simulink model "EMT_ML.before_diagnostic_fixes"  (R2024b)
settings: Solver=ode5  StartTime=0.0  StopTime=200  FixedStep=0.002  RelTol=1e-3
model workspace (MAT data in the model file):
  A = 7.3
  B = 2.71
  C0_shift = 200
  C1_shift = 200
  C2_shift = 200
  Cb = 70
  Cd = 0.6
  EMSInputBus : Simulink.Bus (value not decoded)
  Fb_max = 247500
  JA = 0.4
  JB = 0.4
  JZ = 0.4
  Jc1r2 = 0.01
  Jc3r4 = 0.01
  Jc4 = 0.01
  Je = 2.5
  Jh = 0.01
  Jq1 = 0.01
  Jq2 = 0.01
  Jr1 = 0.01
  Jr3s4 = 0.01
  Js123 = 0.01
  L = 4.472
  NE = [1600 1600 1600 1600 1600 1600 1600 1600 1600 1600 1600 1600 ... (840 elements, 30x28)]
  N_Te = 30
  N_ne = 28
  PE = [0 100.366530527 133.710336161 167.221698607 195.706356687 221.845219395 250.497434286 278.144308305 305.288511886 330.086920096 352.87464656 374.489475338 ... (840 elements, 30x28)]
  PN0 = 0
  Pb_epr = [-45 -45 -40 -30 0 30 40 45 45]
  Pb_max = [0 40 45 45 45]
  Pb_min = [-45 -45 -45 -40 0]
  Pe_ass = 230
  Pe_max = 1103
  Peg = [0 100 120 140 160 180 200 220 240 260 280 300 ... (53 elements, 1x53)]
  R_map = [0.09 0.089 0.09 0.091 0.092 0.093 0.094 0.095 0.096 0.097 0.098]
  SF_C0 = 1.5
  SF_C1 = 1.5
  SF_C2 = 1.5
  SF_Z1 = 1.5
  SF_Z2 = 1.5
  SF_ZD = 1.5
  SOC0 = 60
  SOC_epr = [30 31 50 59 60 61 70 79 80]
  SOC_map = [0 10 20 30 40 50 60 70 80 90 100]
  TA_max_map = [588.855 593.803361345 598.83559322 603.953846154 609.160344828 614.457391304 619.847368421 625.332743363 630.916071429 636.6 642.387272727 648.280733945 ... (115 elements, 1x115)]
  TA_min_map = [-588.855 -593.803361345 -598.83559322 -603.953846154 -609.160344828 -614.457391304 -619.847368421 -625.332743363 -630.916071429 -636.6 -642.387272727 -648.280733945 ... (115 elements, 1x115)]
  TAf = 0
  TB_max_map = [588.855 593.803361345 598.83559322 603.953846154 609.160344828 614.457391304 619.847368421 625.332743363 630.916071429 636.6 642.387272727 648.280733945 ... (115 elements, 1x115)]
  TB_min_map = [-588.855 -593.803361345 -598.83559322 -603.953846154 -609.160344828 -614.457391304 -619.847368421 -625.332743363 -630.916071429 -636.6 -642.387272727 -648.280733945 ... (115 elements, 1x115)]
  TBf = 0
  TE = [0 599 798 998 1168 1324 1495 1660 1822 1970 2106 2235 ... (840 elements, 30x28)]
  TS_A = 0.2
  TS_B = 0.2
  TS_C0 = 0.2
  TS_C1 = 0.2
  TS_C2 = 0.2
  TS_Z = 0.2
  TS_Z1 = 0.2
  TS_Z2 = 0.2
  TS_ZD = 0.2
  TZ_max_map = [537.13125 540.509433962 543.930379747 547.394904459 550.903846154 554.458064516 558.058441558 561.705882353 565.401315789 569.145695364 572.94 576.785234899 ... (131 elements, 1x131)]
  TZ_min_map = [-537.13125 -540.509433962 -543.930379747 -547.394904459 -550.903846154 -554.458064516 -558.058441558 -561.705882353 -565.401315789 -569.145695364 -572.94 -576.785234899 ... (131 elements, 1x131)]
  TZf = 0
  T_generator = [0 185 493.333333333 801.666666667 1110 1418.33333333 1726.66666667]
  T_motor = [0 185 493.333333333 801.666666667 1110 1418.33333333 1726.66666667]
  Te_map = [0 599 798 998 1168 1324 1495 1660 1822 1970 2106 2235 ... (30 elements, 1x30)]
  Te_max = 2754
  Te_max_map = [1168 1324 1495 1660 1822 1970 2106 2235 2355 2458 2543 2606 ... (28 elements, 1x28)]
  Te_start = 1600
  Tef = 100
  Teg = [0 596.8125 636.6 718.741935484 799.916230366 859.41 954.422788606 954.9 996.417391304 1078.98305085 1114.05 1169.26530612 ... (53 elements, 1x53)]
  Temax = 998
  Time = [0 0.1 0.2 0.3 0.4 0.5 0.6 0.7 0.8 0.9 1 1.1 ... (2001 elements, 1x2001)]
  Time_ele = [0 4 8 12 16 20 24 28 32 36 40 44 ... (401 elements, 1x401)]
  Time_fg = [0 2 4 6 8 10 12 14 16 18 20 22 ... (801 elements, 1x801)]
  Tmax_C0 = 2754
  Tmax_C1 = 3505.25455609
  Tmax_C2 = 3505.25455609
  Tmax_Z1 = 5584.80955498
  Tmax_Z2 = 16307.6439005
  Tmax_ZD = 3855.6
  Ts_e = 0.1
  Uoc_map = [814.5 917 933.25 945.75 958.25 969.25 978 985.25 993.25 1003.25 1050]
  V_Shift12 = 32
  V_Shift21 = 25
  V_Start = 10
  Voltage0 = 900
  Voltage_epr = [750 760 900 1000 1050]
  Y_engine = 0.955
  Yc = 0.98
  Yh = 0.96
  Yo = 0.92
  Yq = 0.94
  Z1_shift = 200
  Z2_shift = 200
  a11 = 1.54241568346
  a11_L = 1.54241568346
  a12 = -3.86074191629
  a12_L = 2.43173643789
  a21 = -1.04963112005
  a22 = 2.46948356808
  b11 = 0
  b11_L = 0
  b12 = 3.33
  b12_L = 7.8036
  b21 = 2.23571428571
  b22 = -2.13
  c11 = -0.648333656565
  c12 = 0
  c21 = -0.648333656565
  c22 = 0.680511182109
  controller_id = 1
  controller_name = 'Existing heuristic-grid EMS'
  cycle_grade = [0 0 0 0 0 0 0 0 0 0 0 0 ... (2001 elements, 1x2001)]
  cycle_road = [0.045 0.045 0.045 0.045 0.045 0.045 0.045 0.045 0.045 0.045 0.045 0.045 ... (2001 elements, 1x2001)]
  cycle_steering = [0 0 0 0 0 0 0 0 0 0 0 0 ... (2001 elements, 1x2001)]
  cycle_time = [0 0.1 0.2 0.3 0.4 0.5 0.6 0.7 0.8 0.9 1 1.1 ... (2001 elements, 1x2001)]
  d11 = -0.751666343435
  d12 = 0.3003003003
  d21 = -0.751666343435
  d22 = 0.319488817891
  e11 = -1.54241568346
  e12 = 0
  e21 = 1.04963112005
  e22 = -2.23571428571
  eff_generator = [0.8 0.8 0.79 0.79 0.76 0.74 0.72 0.8 0.85 0.88 0.85 0.8 ... (84 elements, 7x12)]
  eff_motor = [0.8 0.8 0.79 0.79 0.76 0.74 0.72 0.8 0.85 0.88 0.85 0.8 ... (84 elements, 7x12)]
  ele_map = [10 11.46 14.13 19.24 20.94 23.21 20.29 20.23 22.28 17.66 16.24 18.95 ... (401 elements, 1x401)]
  ems_runtime_config : object (value not decoded)
  f11 = -3.86074191629
  f12 = 3.33
  f21 = 2.46948356808
  f22 = -2.13
  fg = 0.045
  fg_map = [0.0125 0.0215 0.0332 0.0452 0.0525 0.0589 0.0584 0.0592 0.0621 0.0576 0.055 0.0572 ... (801 elements, 1x801)]
  fuel_gpkwh = [269.874826377 269.874826377 260.084605263 254.895150301 249.802821062 244.062054381 234.972466555 226.630558735 223.93243551 227.612775381 231.379615385 228.983738255 ... (840 elements, 30x28)]
  fuel_map = [269.874826377 269.874826377 260.084605263 254.895150301 249.802821062 244.062054381 234.972466555 226.630558735 223.93243551 227.612775381 231.379615385 228.983738255 ... (840 elements, 30x28)]
  fuel_map_N = [269.874826377 269.874826377 260.084605263 254.895150301 249.802821062 nan nan nan nan nan nan nan ... (840 elements, 30x28)]
  i = 28
  ic = 4.42
  iq = 1.4
  it = 4
  j = 30
  k1 = 2.13
  k2 = 2.13
  k3 = 2.33
  k4 = 1.92
  kh = 2.88
  kq = 2.17
  kt = 1.83
  mass = 45000
  miu_max = 0.8
  nA_map = [-6000 -5950 -5900 -5850 -5800 -5750 -5700 -5650 -5600 -5550 -5500 -5450 ... (115 elements, 1x115)]
  nA_max = 6000
  nA_min = -6000
  nB_map = [-6000 -5950 -5900 -5850 -5800 -5750 -5700 -5650 -5600 -5550 -5500 -5450 ... (115 elements, 1x115)]
  nB_max = 6000
  nB_min = -6000
  nB_start = 0
  nZ_map = [-8000 -7950 -7900 -7850 -7800 -7750 -7700 -7650 -7600 -7550 -7500 -7450 ... (131 elements, 1x131)]
  nZ_max = 8000
  nZ_min = -8000
  n_generator = [0 318.5 796.25 1274 1751.75 2229.5 2707.25 3185 3662.75 4140.5 4618.25 7007]
  n_motor = [0 318.5 796.25 1274 1751.75 2229.5 2707.25 3185 3662.75 4140.5 4618.25 7007]
  ne_idl = 3000
  ne_map = [1600 1700 1800 1900 2000 2100 2200 2300 2400 2500 2600 2700 ... (28 elements, 1x28)]
  ne_max = 4200
  ne_min = 1600
  ne_start = 200
  neg = [1600 1600 1800 1860 1910 2000 2001 2200 2300 2301 2400 2450 ... (53 elements, 1x53)]
  no_Shift12 = 1589.43589002
  no_Shift21 = 1241.74678908
  rz = 0.318
  startup_feedback_delay_s = 0.002
  startup_power_share = 0.5
  startup_speed_regularizer_rpm = 100
  v_cyc = [0 0 0 0 0 0 0 0 0 0 0 0 ... (2001 elements, 1x2001)]
  voltage_HighA = 1050
  voltage_HighB = 1050
  voltage_HighZ = 1050
  voltage_LowA = 750
  voltage_LowB = 750
  voltage_LowZ = 750
symbols that are objects in the model workspace (value not decoded): ems_runtime_config
undefined symbols (not defined in the file or in its folder): sigbuilder_block
libraries: fl_lib x82, nesl_utility x55, simulink x49, sdl_lib x10, simulink_need_slupdate x6, powerlib_extras x1
(part 7 of 7)

== system EMT_ML.before_diagnostic_fixes/Control Unit/Control/Power Distribution/Feasible Control Range/State Calculation/Speed/Z ==
  s : Inport
  ne : Inport  Port=2
  no : Inport  Port=3
  Multiport Switch1 : MultiPortSwitch  Inputs=4  SaturateOnIntegerOverflow=off  InputSameDT=off
  Mux2 : Mux  Inputs=2
  Subsystem2 : Subsystem
  Subsystem3 : Subsystem
  Subsystem4 : Subsystem
  Subsystem5 : Subsystem
  nAnB : Outport
  wires:
  no/1 -> Mux2/2
  ne/1 -> Mux2/1
  s/1 -> Multiport Switch1/1
  Multiport Switch1/1 -> nAnB/1
  Mux2/1 -> Subsystem3/1(neno), Subsystem4/1(neno), Subsystem5/1(neno), Subsystem2/1(neno)
  Subsystem5/1(nAnB) -> Multiport Switch1/4
  Subsystem4/1(nAnB) -> Multiport Switch1/3
  Subsystem3/1(nAnB) -> Multiport Switch1/2
  Subsystem2/1(nAnB) -> Multiport Switch1/5

== system EMT_ML.before_diagnostic_fixes/Control Unit/Control/Power Distribution/Feasible Control Range/State Predition/Z/ne Range ==
  stage : Inport
  no : Inport  Port=2
  Demux : Demux  Outputs=2
  Multiport Switch : MultiPortSwitch  Inputs=4  SaturateOnIntegerOverflow=off  InputSameDT=off
  Subsystem : Subsystem
  Subsystem1 : Subsystem
  Subsystem2 : Subsystem
  Subsystem3 : Subsystem
  Subsystem4 : Subsystem
  ne_max : Outport
  ne_min : Outport  Port=2
  wires:
  Subsystem4/1(ne) -> Multiport Switch/5
  Subsystem3/1(1) -> Multiport Switch/1
  Subsystem/1(ne) -> Multiport Switch/2
  Subsystem1/1(ne) -> Multiport Switch/3
  Subsystem2/1(ne) -> Multiport Switch/4
  Multiport Switch/1 -> Demux/1
  Demux/1 -> ne_max/1
  Demux/2 -> ne_min/1
  stage/1 -> Subsystem3/1(0)
  no/1 -> Subsystem/1(no), Subsystem4/1(no), Subsystem2/1(no), Subsystem1/1(no)

== system EMT_ML.before_diagnostic_fixes/Control Unit/Control/Prepare Stage/motorA torque/TA_com1/Subsystem1/Subsystem ==
  dnA : Inport
  Abs : Abs  SaturateOnIntegerOverflow=off
  Constant1 : Constant  Value=min(TA_min_map)
  Constant2 : Constant  Value=max(TA_max_map)
  PID Controller2 : simulink_need_slupdate/PID Controller  P=10  I=0.1  D=1
  Switch1 : Switch  Criteria=u2 > Threshold  Threshold=1000  SaturateOnIntegerOverflow=off  InputSameDT=off
  Switch2 : Switch  Criteria=u2 > Threshold  SaturateOnIntegerOverflow=off  InputSameDT=off
  TA : Outport
  wires:
  dnA/1 -> PID Controller2/1, Switch2/2, Abs/1
  PID Controller2/1 -> Switch1/3
  Switch1/1 -> TA/1
  Abs/1 -> Switch1/2
  Switch2/1 -> Switch1/1
  Constant1/1 -> Switch2/3
  Constant2/1 -> Switch2/1

== system EMT_ML.before_diagnostic_fixes/Control Unit/Control/Power Distribution/Feasible Control Range/State Calculation/Speed/Z/Subsystem2 ==
  neno : Inport
  Mux2 : Mux  Inputs=2
  ne_max1 : Fcn  Expr=b11/kt*u(1)+b12*u(2)
  ne_max3 : Fcn  Expr=a11_L*u(1)+a12*u(2)
  nAnB : Outport
  wires:
  ne_max3/1 -> Mux2/1
  ne_max1/1 -> Mux2/2
  neno/1 -> ne_max1/1, ne_max3/1
  Mux2/1 -> nAnB/1

== system EMT_ML.before_diagnostic_fixes/Control Unit/Control/Power Distribution/Feasible Control Range/State Calculation/Speed/Z/Subsystem3 ==
  neno : Inport
  Mux2 : Mux  Inputs=2
  ne_max1 : Fcn  Expr=b11*u(1)+b12*u(2)
  ne_max3 : Fcn  Expr=a11*u(1)+a12*u(2)
  nAnB : Outport
  wires:
  ne_max3/1 -> Mux2/1
  ne_max1/1 -> Mux2/2
  neno/1 -> ne_max1/1, ne_max3/1
  Mux2/1 -> nAnB/1

== system EMT_ML.before_diagnostic_fixes/Control Unit/Control/Power Distribution/Feasible Control Range/State Calculation/Speed/Z/Subsystem4 ==
  neno : Inport
  Mux2 : Mux  Inputs=2
  ne_max1 : Fcn  Expr=b11*u(1)+b12*u(2)
  ne_max3 : Fcn  Expr=a11*u(1)+a12*u(2)
  nAnB : Outport
  wires:
  Mux2/1 -> nAnB/1
  neno/1 -> ne_max3/1, ne_max1/1
  ne_max1/1 -> Mux2/2
  ne_max3/1 -> Mux2/1

== system EMT_ML.before_diagnostic_fixes/Control Unit/Control/Power Distribution/Feasible Control Range/State Calculation/Speed/Z/Subsystem5 ==
  neno : Inport
  Mux2 : Mux  Inputs=2
  ne_max1 : Fcn  Expr=b21*u(1)+b22*u(2)
  ne_max3 : Fcn  Expr=a21*u(1)+a22*u(2)
  nAnB : Outport
  wires:
  ne_max3/1 -> Mux2/1
  ne_max1/1 -> Mux2/2
  neno/1 -> ne_max1/1, ne_max3/1
  Mux2/1 -> nAnB/1

== system EMT_ML.before_diagnostic_fixes/Control Unit/Control/Power Distribution/Feasible Control Range/State Predition/Z/ne Range/Subsystem ==
  no : Inport
  Mux2 : Mux  Inputs=2
  ne_max : Fcn  Expr=(nA_max-a12*u)/a11
  ne_min : Fcn  Expr=(nA_min-a12*u)/a11
  ne : Outport
  wires:
  no/1 -> ne_min/1, ne_max/1
  ne_max/1 -> Mux2/1
  Mux2/1 -> ne/1
  ne_min/1 -> Mux2/2

== system EMT_ML.before_diagnostic_fixes/Control Unit/Control/Power Distribution/Feasible Control Range/State Predition/Z/ne Range/Subsystem1 ==
  no : Inport
  Mux2 : Mux  Inputs=2
  ne_max : Fcn  Expr=(nB_max-b22*u)/b21
  ne_min : Fcn  Expr=(nA_min-a12*u)/a11
  ne : Outport
  wires:
  ne_min/1 -> Mux2/2
  Mux2/1 -> ne/1
  ne_max/1 -> Mux2/1
  no/1 -> ne_max/1, ne_min/1

== system EMT_ML.before_diagnostic_fixes/Control Unit/Control/Power Distribution/Feasible Control Range/State Predition/Z/ne Range/Subsystem2 ==
  no : Inport
  MinMax1 : MinMax  Inputs=2
  MinMax2 : MinMax  Function=max  Inputs=2
  Mux2 : Mux  Inputs=2
  ne_max1 : Fcn  Expr=(nA_min-a22*u)/a21
  ne_max2 : Fcn  Expr=(nB_max-b22*u)/b21
  ne_min1 : Fcn  Expr=(nA_max-a22*u)/a21
  ne_min2 : Fcn  Expr=(nB_min-b22*u)/b21
  ne : Outport
  wires:
  MinMax2/1 -> Mux2/2
  MinMax1/1 -> Mux2/1
  no/1 -> ne_max1/1, ne_min1/1, ne_min2/1, ne_max2/1
  Mux2/1 -> ne/1
  ne_max1/1 -> MinMax1/1
  ne_max2/1 -> MinMax1/2
  ne_min1/1 -> MinMax2/1
  ne_min2/1 -> MinMax2/2

== system EMT_ML.before_diagnostic_fixes/Control Unit/Control/Power Distribution/Feasible Control Range/State Predition/Z/ne Range/Subsystem3 ==
  0 : Inport
  Constant : Constant
  Constant1 : Constant  Value=4
  MinMax : MinMax  Function=max  Inputs=2
  MinMax1 : MinMax  Inputs=2
  1 : Outport
  wires:
  0/1 -> MinMax/1
  Constant/1 -> MinMax/2
  MinMax/1 -> MinMax1/1
  Constant1/1 -> MinMax1/2
  MinMax1/1 -> 1/1

== system EMT_ML.before_diagnostic_fixes/Control Unit/Control/Power Distribution/Feasible Control Range/State Predition/Z/ne Range/Subsystem4 ==
  no : Inport
  Mux2 : Mux  Inputs=2
  ne_max : Fcn  Expr=(nA_max-a12_L*u)/a11_L
  ne_min : Fcn  Expr=(nA_min-a12_L*u)/a11_L
  ne : Outport
  wires:
  ne_min/1 -> Mux2/2
  Mux2/1 -> ne/1
  ne_max/1 -> Mux2/1
  no/1 -> ne_max/1, ne_min/1

== matlab function EMT_ML.before_diagnostic_fixes/Control Unit/Control/Power Distribution/Optimal Power Distribution/Optimization  ==
  data: u input; y output
function y = fcn(u)
%#codegen
Pe_com=u(1);pedal=u(2);ZD=u(3);stage=u(4);ne_act=u(5);ne_max=u(6);ne_min=u(7);
no_act=u(8);Te_max=u(9);Te_min=u(10);TA_max=u(11);TA_min=u(12);TB_max=u(13);
TB_min=u(14);PN_com=u(15);PN_max=u(16);PN_min=u(17);PZ_com=u(18);sd_ne=u(19);
%转速转矩关系
a11=1.5424;a12=-3.8607;%EVT1模式下nA表达式的系数nA=a11*ne+a12*no
a11_L=1.5424;a12_L=2.4317;%EVT1_L模式下nA表达式的系数nA=a11_L*ne+a12_L*no
b11=0;b12=3.3300;%EVT1模式下nB表达式的系数nB=b11*ne+b12*no
b11_L=0;b12_L=7.8036;%EVT1模式下nB表达式的系数nB=b11*ne+b12*no
a21=-1.0496;a22=2.4695;%EVT2模式下nA表达式的系数nA=a21*ne+a22*no
b21=2.2357;b22=-2.1300;%EVT2模式下nB表达式的系数nB=b21*ne+b22*no
e11=-1.5424;e12=0;%EVT1模式下Te表达式的系数Te=e11*TA+e12*TB
f11=-3.8607;f12=3.3300;%EVT1模式下To表达式的系数To=f11*TA+f12*TB
e21=1.0496;e22=-2.2357;%EVT2模式下Te表达式的系数Te=e21*TA+e22*TB
f21=2.4695;f22=-2.1300;%EVT2模式下To表达式的系数To=f21*TA+f22*TB
kq=2.17;YE=0.75;YA=0.8;YB=0.8;%平均效率
if pedal>0.99&&no_act<49.67*50
    TA_max=1.5*TA_max;TA_min=1.5*TA_min;
    TB_max=1.5*TB_max;TB_min=1.5*TB_min;
else
end
if stage<3
    nA=a11*ne_act+a12*no_act;
    nB=b11*ne_act+b12*no_act;
elseif stage<4
    nA=a21*ne_act+a22*no_act;
    nB=b21*ne_act+b22*no_act;
else
    nA=a11_L*ne_act+a12_L*no_act;
    nB=b11_L*ne_act+b12_L*no_act;
end
%发动机燃油经济性曲线
Peg=[0,100,120,140,160,180,200,220,240,260,280,300,320,340,360,380,400,420,440,460,480,500,520,540,560,580,600,620,640,660,680,700,720,740,760,780,800,820,840,860,880,900,920,940,960,980,1000,1020,1040,1060,1080,1100,1200];
neg=[1600,1600,1800,1860,1910,2000,2001,2200,2300,2301,2400,2450,2610,2611,2612,2613,2700,2701,2702,2730,2790,2880,2900,2901,2902,2903,3200,3201,3202,3203,3204,3205,3206,3207,3300,3301,3302,3310,3350,3390,3420,3500,3501,3700,3701,3702,3760,3761,3810,4180,4200,4200,4200];
Pe_com=min(Pe_com,max(Peg));
Pe_com=max(Pe_com,min(Peg));
ne_ref=interp1(Peg,neg,Pe_com);
ne_idl=3000;%发动机启动转速
V_Shift12=32;%EVT1到EVT2的换段车速(km/h)
V_Shift21=25;%EVT2到EVT1的换段车速(km/h)
alpha=max(pedal,0);
V_Shift12=V_Shift12-5*(1-alpha);
V_Shift21=V_Shift21+5*alpha;
if stage<3&&no_act>49.67*(V_Shift12-2)
    ne_ref=max(2.442*no_act,ne_ref);
elseif stage>1&&no_act<49.67*(V_Shift21+2)
    ne_ref=min(2.442*no_act,ne_ref);
elseif pedal<0
    ne_ref=2.442*no_act;   
else
end
if pedal>0.8&&ne_max<4200&&no_act<49.67*10
    ne_max=ne_max-500;
else
end
ne_min=max(ne_idl,ne_min);ne_max=min(4200,ne_max);
ne_min=max(ne_act-100,ne_min);ne_max=min(ne_act+500,ne_max);
ne_ref=max(ne_ref,ne_min);ne_ref=min(ne_ref,ne_max);
ne_ref0=ne_ref;
if pedal>0
    ne_ref=ne_ref+sd_ne;
else
end
% x_ne=[-500 -200 -100 -50 0 50 100 200 500];
% x_Te=[0.1 0.2 0.5 0.8 1 1.5 2.0 5.0 10];
x_ne=[-200 0 200];
x_Te=[0.6 1 2.0];
dne=ne_ref-ne_act;dne=min(dne,200);dne=max(dne,-200);
x_ne=interp1(x_ne,x_Te,dne);
if ne_act==0
    Te_ref=Te_max;
else
    Te_ref=9549*Pe_com/ne_act;
end
Te_ref=max(Te_ref,200);
Te_ref=x_ne*Te_ref;
Te_ref=max(Te_ref,Te_min);Te_ref=min(Te_ref,Te_max);
Te1=linspace(Te_ref,Te_min,10);Te2=linspace(Te_ref,Te_max,10);
Te=[Te1 Te2];L_Te=length(Te);
TA=linspace(TA_min,TA_max,20);L_TA=length(TA);
TB=linspace(TB_min,TB_max,20);L_TB=length(TB);
TA0=zeros(1,L_TA*L_TB);TB0=zeros(1,L_TA*L_TB);
for i=1:L_TA
    for j=1:L_TB
        TA0((j-1)*L_TA+i)=TA(i);
        TB0((j-1)*L_TA+i)=TB(j);
    end
end
TA=TA0;TB=TB0;
if ZD==1
    if stage==3
        Tef=(e21.*TA+e22.*TB);
        To=(f21.*TA+f22.*TB);
    else
        Tef=(e11.*TA+e12.*TB);
        To=(f11.*TA+f12.*TB);
    end
else
    if stage==3
        Tef=(e21.*TA+e22.*TB)/kq;
        To=(f21.*TA+f22.*TB)/kq;
    else
        Tef=(e11.*TA+e12.*TB)/kq;
        To=(f11.*TA+f12.*TB)/kq;
    end
end
Tef=Tef*YE;
PA=TA*nA/9549;PB=TB*nB/9549;
PN=PA.*YA.^sign(-PA)+PB.*YB.^sign(-PB);
PN_com=PN_com-PZ_com;
TA_ref=0;TB_ref=0;
J0=1e10;NN_Te=0;
NN_ne=zeros(L_Te,L_TA*L_TB);
NN_PN0=zeros(L_Te,L_TA*L_TB);
NN_PN1=zeros(L_Te,L_TA*L_TB);
for i=1:L_Te    
    for j=1:L_TA*L_TB
        if (PN(j)<3*PN_min&&PN(j)-PN_com<3*PN_min)||(PN(j)>3*PN_max&&PN(j)-PN_com>3*PN_max)
            continue;
        else
        end
        NN_PN0(i,j)=1;         
        if dne>10
            if Tef(j)*x_ne>Te(i)
                continue;
            else
            end     
        elseif dne<-10
            if Tef(j)*x_ne<Te(i)
                continue;
            else
            end
        else
        end
        NN_ne(i,j)=1;
        if PN(j)-PN_com<3*PN_min||PN(j)-PN_com>3*PN_max
            continue;
        else
        end
        NN_PN1(i,j)=1;
        if PN(j)-PN_com<PN_min||PN(j)-PN_com>PN_max
            continue;
        else
        end
        if PN_com>0
            if PN(j)<0
                continue;
            else
            end
        elseif PN_com<0 
            if PN(j)>0
                continue;
            else
            end
        else
        end
        if pedal>=0.9
            J1=0;
        elseif pedal<=0
            J1=PN(i);
        else
            J1=abs(PN(j)-PN_com);
        end
        if pedal<=0
            J2=0;
        else
            J2=-To(j)*ne_ref/9549;
        end
        J=J1+J2;
        if J<J0
            J0=J;
            Te_ref=Te(i);TA_ref=TA(j);TB_ref=TB(j);
            NN_Te=1;
        else
        end
    end
    if NN_Te==1
        break;
    else
    end
    for j=1:L_TA*L_TB
        if NN_PN1(i,j)==0
            continue;
        else
        end
        if pedal>=0.9
            J1=0;
        elseif pedal<=0
            J1=PN(i);
        else
            J1=abs(PN(j)-PN_com);
        end
        if pedal<=0
            J2=0;
        else
            J2=-To(j)*ne_ref/9549;
        end
        J=J1+J2;
        if J<J0
            J0=J;
            Te_ref=Te(i);TA_ref=TA(j);TB_ref=TB(j);
            NN_Te=1;
        else
        end
    end
    if NN_Te==1
        break;
    else
    end
end
if NN_Te==0
    for i=1:L_Te    
        for j=1:L_TA*L_TB
            if NN_ne(i,j)==0
                continue;
            else
            end
            if PN_com<0
                if PN(j)-PN_com>3*PN_max
                    continue;
                else
                end
                J1=PN(j);
            else
                if PN(j)-PN_com<3*PN_min
                    continue;
                else
                end
                J1=-PN(j);
            end
            if pedal<=0
                J2=0;
            else
                J2=-To(j)*ne_ref/9549;
            end
            J=100*J1+J2;
            if J<J0
                J0=J;
                Te_ref=Te(i);TA_ref=TA(j);TB_ref=TB(j);

            else
            end 
        end
    end
else
end
if NN_Te==0
    if ne_ref>ne_act
        Te_ref=Te_max;
    else
        Te_ref=Te_min;
    end
    for j=1:L_TA*L_TB
        if  NN_PN0(i,j)==0
            continue;
        else
        end
        if ne_ref>ne_act
            J1=Tef(j);
        else
            J1=-Tef(j);
        end
        if pedal<=0
            J2=0;
        else
            J2=-To(j);
        end
        J=100*J1+J2;
        if J<J0
            J0=J;
            Te_ref=Te(i);TA_ref=TA(j);TB_ref=TB(j);
            NN_Te=1;
        else
        end 
    end
else
end
if NN_Te==0
    for i=1:L_Te    
        for j=1:L_TA*L_TB
            if dne>10
                if Tef(j)*x_ne>Te(i)
                    continue;
                else
                end     
            elseif dne<-10
                if Tef(j)*x_ne<Te(i)
                    continue;
                else
                end
            else
            end
            if PN(j)<PN_min
                J1=-PN(j);
            elseif PN(j)>PN_max
                J1=PN(j);
            else
                J1=abs(PN(j)-PN_com);
            end            
            if pedal<=0
                J2=0;
            else
                J2=-To(j)*ne_ref/9549;
            end
            if ne_ref>ne_act
                J3=Tef(j)*ne_ref/9549;
            else
                J3=-Tef(j)*ne_ref/9549;
            end
            J=J1+J2+100*J3;
            if J<J0
                J0=J;
                Te_ref=Te(i);TA_ref=TA(j);TB_ref=TB(j);
                NN_Te=1;
            else
            end 
        end
    end
else
end
if NN_Te==0
    if ne_ref>ne_act
        Te_ref=Te_max;
    else
        Te_ref=Te_min;
    end
    for j=1:L_TA*L_TB
        if PN(j)<3*PN_min&&PN(j)-PN_com<3*PN_min
            J1=-PN(j);
        elseif PN(j)>3*PN_max&&PN(j)-PN_com>3*PN_max
            J1=PN(j);
        else
            J1=abs(PN(j)-PN_com);
        end            
        if pedal<=0
            J2=0;
        else
            J2=-To(j)*ne_ref/9549;
        end
        J=100*J1+J2;
        if J<J0
            J0=J;
            Te_ref=Te(i);TA_ref=TA(j);TB_ref=TB(j);
        else
        end 
    end
else
end
ne_ref=ne_ref0;
y=[ne_ref Te_ref TA_ref TB_ref];
